simulink library "Lib_Piccolo"  (R2018b)
settings: Solver=VariableStepAuto  StartTime=0.0  StopTime=10.0  RelTol=1e-3
values from neighbouring files (symbols this model uses):
  AccelErrInt2Brakes = 0.15    [SimulationControlConfig16P.m]    (also in SimulationControlConfig16P_LEGACY.m; SimulationControlConfigTAILLESS.m = 0.2; SimulationControlConfigUTAIL.m = 0.2)
  AileronMax = 25    [SimulationControlConfig16P.m]    (also in SimulationControlConfig16P_LEGACY.m; SimulationControlConfigTAILLESS.m; SimulationControlConfigUTAIL.m)
  AileronPower = 0.00268    [SimulationControlConfig16P.m]    (also in SimulationControlConfig16P_LEGACY.m; SimulationControlConfigTAILLESS.m; SimulationControlConfigUTAIL.m)
  AileronSurfaceMax = 45    [SimulationControlConfig16P.m]    (also in SimulationControlConfig16P_LEGACY.m)
  AileronTrim = 0    [SimulationControlConfig16P.m]    (also in SimulationControlConfig16P_LEGACY.m; SimulationControlConfigTAILLESS.m; SimulationControlConfigUTAIL.m)
  Alt = 1000 + TerrainHeight    [SimulationStateConfig.m]
  AltCruise_m = testPlans(testIndx).terrainElevation * 0.3048 + 200    [SimulationControlConfig16P.m]    (also in SimulationControlConfigTAILLESS.m = 1083; SimulationControlConfigUTAIL.m = testPlans(testIndx).terrainElevation * 0.3048 + 152)
  AltitudeRate2PitchCmdIntegratorInit = 0.1    [SimulationControlPre.m]
  AltMax = 10000    [SimulationControlConfig16P.m]    (also in SimulationControlConfig16P_LEGACY.m; SimulationControlConfigTAILLESS.m; SimulationControlConfigUTAIL.m)
  AltMaxAccel = 1.25    [SimulationControlConfig16P.m]    (also in SimulationControlConfig16P_LEGACY.m = 0.9; SimulationControlConfigTAILLESS.m = 1.7; SimulationControlConfigUTAIL.m = 2)
  AltMin = 0    [SimulationControlConfig16P.m]    (also in SimulationControlConfig16P_LEGACY.m; SimulationControlConfigTAILLESS.m; SimulationControlConfigUTAIL.m)
  AltRateCmd2Pitch = 0.50    (= 0.5)    [SimulationControlConfig16P.m]    (also in SimulationControlConfig16P_LEGACY.m = 0.6; SimulationControlConfigTAILLESS.m = 0.2; SimulationControlConfigUTAIL.m = 0.3)
  AltRateError2Pitch = 0.40    (= 0.4)    [SimulationControlConfig16P.m]    (also in SimulationControlConfig16P_LEGACY.m; SimulationControlConfigTAILLESS.m = 0.55; SimulationControlConfigUTAIL.m = 0.55)
  AltRateErrorInt2Pitch = 0.50    (= 0.5)    [SimulationControlConfig16P.m]    (also in SimulationControlConfig16P_LEGACY.m = 0.45; SimulationControlConfigTAILLESS.m; SimulationControlConfigUTAIL.m = 0.75)
  AltRateLpfCutOff = 3    [SimulationControlConfig16P.m]    (also in SimulationControlConfig16P_LEGACY.m; SimulationControlConfigTAILLESS.m = 2; SimulationControlConfigUTAIL.m = 2)
  AutoNosegear2Rudder = 26    [SimulationControlConfig16P.m]    (also in SimulationControlConfig16P_LEGACY.m; SimulationControlConfigTAILLESS.m = 25.2; SimulationControlConfigUTAIL.m = 14)
  b = 5.54    [SimulationControlConfig16P.m]    (also in SimulationControlConfig16P_LEGACY.m; SimulationControlConfigTAILLESS.m = 2.37; SimulationControlConfigUTAIL.m = 2.37)
  Bank2AileronIntegratorInit = 0    [SimulationControlPre.m]
  BankMax_User = BankMax_User/180*pi    (= 0.523598775598)    [SimulationControlConfig16P.m]    (also in SimulationControlConfig16P_LEGACY.m; SimulationControlConfigTAILLESS.m = 0.610865238198; SimulationControlConfigUTAIL.m = 0.628318530718)
  baseLegFlaps = 20    [SimulationControlConfig16P.m]    (also in SimulationControlConfig16P_LEGACY.m = 0; SimulationControlConfigTAILLESS.m = 15; SimulationControlConfigUTAIL.m = 10)
  C = GeneticOpt.C    [SimulationCostFunction.m]
  c = Sw/b    (= 0.841696750903)    [SimulationControlConfig16P.m]    (also in SimulationControlConfig16P_LEGACY.m; SimulationControlConfigTAILLESS.m = 0.354008438819; SimulationControlConfigUTAIL.m = 0.354008438819)
  cell2WheelFactorMG = 5.98    [SimulationSensorConfig16P_LEGACY.m]
  cell2WheelFactorNG = 1    [SimulationSensorConfig16P_LEGACY.m]
  cellSatMaxMG = 15000    [SimulationSensorConfig16P.m]    (also in SimulationSensorConfig16P_LEGACY.m; SimulationSensorConfigTAILLESS7P.m; SimulationSensorConfigUTAIL7P.m)
  cellSatMaxNG = 1000    [SimulationSensorConfig16P.m]    (also in SimulationSensorConfig16P_LEGACY.m; SimulationSensorConfigTAILLESS7P.m; SimulationSensorConfigUTAIL7P.m)
  cellSatMinMG = -15000    [SimulationSensorConfig16P.m]    (also in SimulationSensorConfig16P_LEGACY.m; SimulationSensorConfigTAILLESS7P.m; SimulationSensorConfigUTAIL7P.m)
  cellSatMinNG = -1000    [SimulationSensorConfig16P.m]    (also in SimulationSensorConfig16P_LEGACY.m; SimulationSensorConfigTAILLESS7P.m; SimulationSensorConfigUTAIL7P.m)
  CL_Limit = CL_Max    (= 0.54)    [SimulationControlConfig16P.m]    (also in SimulationControlConfig16P_LEGACY.m; SimulationControlConfigTAILLESS.m; SimulationControlConfigUTAIL.m = 0.53)
  CL_Max = 0.54    [SimulationControlConfig16P.m]    (also in SimulationControlConfig16P_LEGACY.m; SimulationControlConfigTAILLESS.m; SimulationControlConfigUTAIL.m = 0.53)
  CL_Max_Nom = 0.465    [SimulationControlConfig16P.m]    (also in SimulationControlConfig16P_LEGACY.m; SimulationControlConfigTAILLESS.m = 0.39; SimulationControlConfigUTAIL.m)
  CL_Min = 0    [SimulationControlConfig16P.m]    (also in SimulationControlConfig16P_LEGACY.m; SimulationControlConfigTAILLESS.m; SimulationControlConfigUTAIL.m)
  ClimbMaxFraction = 0.35    [SimulationControlConfig16P.m]    (also in SimulationControlConfig16P_LEGACY.m = 0.24; SimulationControlConfigTAILLESS.m = 0.19; SimulationControlConfigUTAIL.m = 0.21)
  ClimboutMaxBank = 7.0    (= 7)    [SimulationControlConfig16P.m]    (also in SimulationControlConfig16P_LEGACY.m; SimulationControlConfigTAILLESS.m = 5; SimulationControlConfigUTAIL.m)
  ClimboutTimer = 7.0    (= 7)    [SimulationControlConfig16P.m]    (also in SimulationControlConfig16P_LEGACY.m; SimulationControlConfigTAILLESS.m; SimulationControlConfigUTAIL.m)
  dCl_per_dFlap = 0.005581818    [SimulationControlConfig16P.m]    (also in SimulationControlConfig16P_LEGACY.m = 0; SimulationControlConfigTAILLESS.m = 0; SimulationControlConfigUTAIL.m = 0)
  DecelerationCmd = 3.1    [SimulationControlConfig16P.m]    (also in SimulationControlConfig16P_LEGACY.m; SimulationControlConfigTAILLESS.m = 0.1; SimulationControlConfigUTAIL.m = 0.1)
  DeRotateLogicEndTimer = abs((NoseDownLimit_Deg-1)/DeRotateRamp_Dps)    [SimulationControlConfig16P.m]    (also in SimulationControlConfig16P_LEGACY.m; SimulationControlConfigTAILLESS.m; SimulationControlConfigUTAIL.m)
  DeRotateLogicHoldNoseUpTimer = 0.1    [SimulationControlConfig16P.m]    (also in SimulationControlConfig16P_LEGACY.m; SimulationControlConfigTAILLESS.m; SimulationControlConfigUTAIL.m)
  DeRotateLogicTimerTimeout = 2    [SimulationControlConfig16P.m]    (also in SimulationControlConfig16P_LEGACY.m; SimulationControlConfigTAILLESS.m; SimulationControlConfigUTAIL.m)
  DeRotateLowerCmdSaturation = 0    [SimulationControlConfig16P.m]    (also in SimulationControlConfig16P_LEGACY.m; SimulationControlConfigTAILLESS.m; SimulationControlConfigUTAIL.m)
  DeRotateRamp_Dps = 3    [SimulationControlConfig16P.m]    (also in SimulationControlConfig16P_LEGACY.m; SimulationControlConfigTAILLESS.m = 8; SimulationControlConfigUTAIL.m = 8)
  DeRotateUpperCmdSaturation = 7    [SimulationControlConfig16P.m]    (also in SimulationControlConfig16P_LEGACY.m; SimulationControlConfigTAILLESS.m; SimulationControlConfigUTAIL.m)
  DescentMaxFraction = 0.22    [SimulationControlConfig16P.m]    (also in SimulationControlConfig16P_LEGACY.m = 0.2; SimulationControlConfigTAILLESS.m = 0.17; SimulationControlConfigUTAIL.m = 0.17)
  DesktopSimTerrainOffset_m = 0.406    [SimulationAircraftConfig.m]
  downwindFlaps = 0    [SimulationControlConfig16P.m]    (also in SimulationControlConfig16P_LEGACY.m; SimulationControlConfigTAILLESS.m; SimulationControlConfigUTAIL.m)
  DP_init = 0.5*1.225*V_init^2    [SimulationControlConfig16P.m]    (also in SimulationControlConfig16P_LEGACY.m; SimulationControlConfigTAILLESS.m; SimulationControlConfigUTAIL.m)
  dscNoiseMG = 1    [SimulationSensorConfig16P_LEGACY.m]
  dscNoiseNG = 0.25    [SimulationSensorConfig16P_LEGACY.m]
  DSCnumBits = 24    [SimulationSensorConfig16P.m]    (also in SimulationSensorConfig16P_LEGACY.m; SimulationSensorConfigTAILLESS7P.m; SimulationSensorConfigUTAIL7P.m)
  DSCRangeMaxMG = 15000    [SimulationSensorConfig16P.m]    (also in SimulationSensorConfig16P_LEGACY.m; SimulationSensorConfigTAILLESS7P.m; SimulationSensorConfigUTAIL7P.m)
  DSCRangeMaxNG = 1000    [SimulationSensorConfig16P.m]    (also in SimulationSensorConfig16P_LEGACY.m; SimulationSensorConfigTAILLESS7P.m; SimulationSensorConfigUTAIL7P.m)
  DSCRangeMinMG = -15000    [SimulationSensorConfig16P.m]    (also in SimulationSensorConfig16P_LEGACY.m; SimulationSensorConfigTAILLESS7P.m; SimulationSensorConfigUTAIL7P.m)
  DSCRangeMinNG = -1000    [SimulationSensorConfig16P.m]    (also in SimulationSensorConfig16P_LEGACY.m; SimulationSensorConfigTAILLESS7P.m; SimulationSensorConfigUTAIL7P.m)
  dt = DLLSim.dt    [SimulationTimeStep.m]    (also in SimulationTrim.m = 0.02)
  EarlyTouchdownThreshold = 3.0    (= 3)    [SimulationControlConfig16P.m]    (also in SimulationControlConfig16P_LEGACY.m; SimulationControlConfigTAILLESS.m = 2.2; SimulationControlConfigUTAIL.m = 2.5)
  ElevatorDeflectionRate = 15    [SimulationControlConfig16P.m]    (also in SimulationControlConfig16P_LEGACY.m = 12; SimulationControlConfigTAILLESS.m = 10; SimulationControlConfigUTAIL.m = 12)
  ElevatorMax = 25    [SimulationControlConfig16P.m]    (also in SimulationControlConfig16P_LEGACY.m; SimulationControlConfigTAILLESS.m; SimulationControlConfigUTAIL.m)
  ElevatorPower = -0.002209    [SimulationControlConfig16P.m]    (also in SimulationControlConfig16P_LEGACY.m; SimulationControlConfigTAILLESS.m = -0.002956; SimulationControlConfigUTAIL.m = -0.00205983)
  ElevatorTrim = -3.5    [SimulationControlConfig16P.m]    (also in SimulationControlConfig16P_LEGACY.m; SimulationControlConfigTAILLESS.m = -6; SimulationControlConfigUTAIL.m = -8)
  elevonBias = 0    [SimulationControlConfig16P.m]    (also in SimulationControlConfig16P_LEGACY.m; SimulationControlConfigTAILLESS.m; SimulationControlConfigUTAIL.m)
  Enable_TAS_Protection = 0    [SimulationControlConfig16P.m]    (also in SimulationControlConfig16P_LEGACY.m; SimulationControlConfigTAILLESS.m; SimulationControlConfigUTAIL.m)
  EnableCrossTrackAbort = 1    [SimulationControlConfig16P.m]    (also in SimulationControlConfigTAILLESS.m; SimulationControlConfigUTAIL.m)
  EnergyBandwidth = 0.02    [SimulationControlConfig16P.m]    (also in SimulationControlConfig16P_LEGACY.m; SimulationControlConfigTAILLESS.m = 0.06; SimulationControlConfigUTAIL.m = 0.06)
  EngineLhFuelCut = 0    [SimulationAircraftConfig.m]
  EngineRhFuelCut = 0    [SimulationAircraftConfig.m]
  FastThrottleRate = 0.075    [SimulationControlConfig16P.m]    (also in SimulationControlConfig16P_LEGACY.m = 0.05; SimulationControlConfigTAILLESS.m = 0.1; SimulationControlConfigUTAIL.m = 0.1)
  FilterWarmUpTime = 2    [SimulationSensorConfig16P.m]    (also in SimulationSensorConfig16P_LEGACY.m; SimulationSensorConfigTAILLESS7P.m; SimulationSensorConfigUTAIL7P.m)
  finalApproachFlaps = 20    [SimulationControlConfig16P.m]    (also in SimulationControlConfig16P_LEGACY.m = 0; SimulationControlConfigTAILLESS.m = 22; SimulationControlConfigUTAIL.m = 10)
  FinalDescentSlope_Deg = testPlans(testIndx).descentSlope    [SimulationControlConfig16P.m]    (also in SimulationControlConfig16P_LEGACY.m; SimulationControlConfigTAILLESS.m; SimulationControlConfigUTAIL.m)
  flapMax = 0    [SimulationControlConfig16P.m]    (also in SimulationControlConfig16P_LEGACY.m; SimulationControlConfigTAILLESS.m; SimulationControlConfigUTAIL.m)
  flapRate = 7.5    [SimulationControlConfig16P.m]    (also in SimulationControlConfig16P_LEGACY.m; SimulationControlConfigTAILLESS.m = 6.6; SimulationControlConfigUTAIL.m)
  FlareHeight = 5    [SimulationControlConfig16P.m]    (also in SimulationControlConfig16P_LEGACY.m = 4.8; SimulationControlConfigTAILLESS.m = 2.5; SimulationControlConfigUTAIL.m = 2)
  FlareVerticalRate_mps = -0.4    [SimulationControlConfig16P.m]    (also in SimulationControlConfig16P_LEGACY.m = -0.5; SimulationControlConfigTAILLESS.m = -0.15; SimulationControlConfigUTAIL.m = -0.15)
  Fp_Aileron = 0.55*2*pi*RollRateLpfCutoff*dt    [SimulationControlConfig16P.m]    (also in SimulationControlConfig16P_LEGACY.m; SimulationControlConfigTAILLESS.m; SimulationControlConfigUTAIL.m)
  Fp_Alt = 0.55*AltBandwidth    (= 0.099)    [SimulationControlConfig16P.m]    (also in SimulationControlConfig16P_LEGACY.m; SimulationControlConfigTAILLESS.m = 0.587477826221; SimulationControlConfigUTAIL.m = 0.69115038379)
  Fp_AltRate = 0.55*2*pi*AltRateLpfCutOff*dt    [SimulationControlConfig16P.m]    (also in SimulationControlConfig16P_LEGACY.m; SimulationControlConfigTAILLESS.m; SimulationControlConfigUTAIL.m)
  Fp_Elevator = 0.55*2*pi*PitchRateLpfCutoff*dt    [SimulationControlConfig16P.m]    (also in SimulationControlConfig16P_LEGACY.m; SimulationControlConfigTAILLESS.m; SimulationControlConfigUTAIL.m)
  Fp_Energy = 0.55*2*pi*EnergyBandwidth    (= 0.069115038379)    [SimulationControlConfig16P.m]    (also in SimulationControlConfig16P_LEGACY.m; SimulationControlConfigTAILLESS.m = 0.207345115137; SimulationControlConfigUTAIL.m = 0.207345115137)
  Fp_Energy2 = 0.55*2*pi*EnergyBandwidth*dt    [SimulationControlConfig16P.m]    (also in SimulationControlConfig16P_LEGACY.m; SimulationControlConfigTAILLESS.m; SimulationControlConfigUTAIL.m)
  Fp_Pitch = 0.55*2*pi*PitchBandwidth    (= 2.76460153516)    [SimulationControlConfig16P.m]    (also in SimulationControlConfig16P_LEGACY.m = 3.11017672705; SimulationControlConfigTAILLESS.m = 3.80132711084; SimulationControlConfigUTAIL.m = 2.41902634326)
  Fp_Pitch_2 = 0.55*2*pi*PitchBandwidth*dt    [SimulationControlConfig16P.m]    (also in SimulationControlConfig16P_LEGACY.m; SimulationControlConfigTAILLESS.m; SimulationControlConfigUTAIL.m)
  Fp_Roll = RollBandwidth^2    (= 1)    [SimulationControlConfig16P.m]    (also in SimulationControlConfig16P_LEGACY.m = 1.44; SimulationControlConfigTAILLESS.m; SimulationControlConfigUTAIL.m)
  Fp_Rudder = 0.55*2*pi*YawRateLpfCutoff*dt    [SimulationControlConfig16P.m]    (also in SimulationControlConfig16P_LEGACY.m; SimulationControlConfigTAILLESS.m; SimulationControlConfigUTAIL.m)
  Fp_TAS = 0.55*2*pi*TASBandwidth    (= 0.103672557568)    [SimulationControlConfig16P.m]    (also in SimulationControlConfig16P_LEGACY.m; SimulationControlConfigTAILLESS.m = 0.172787595947; SimulationControlConfigUTAIL.m = 0.172787595947)
  Fp_TAS_Filter = 2*pi*TasLpfCutoff*dt    [SimulationControlConfig16P.m]    (also in SimulationControlConfig16P_LEGACY.m; SimulationControlConfigTAILLESS.m; SimulationControlConfigUTAIL.m)
  Fp_Turn = 0.55*2*pi*TurnErrLPFcutoff    (= 0.0345575191895)    [SimulationControlConfig16P.m]    (also in SimulationControlConfig16P_LEGACY.m; SimulationControlConfigTAILLESS.m = 0.172787595947; SimulationControlConfigUTAIL.m = 0.172787595947)
  Fp_TurnDerr = 0.55*2*pi*TurnDerivativeLPFcutoff    (= 0.0345575191895)    [SimulationControlConfig16P.m]    (also in SimulationControlConfig16P_LEGACY.m; SimulationControlConfigTAILLESS.m = 0.172787595947; SimulationControlConfigUTAIL.m = 0.172787595947)
  FTV = 3    [SimulationAircraftConfig.m]
  ftvStaticPositionError = 1/1.18    (= 0.847457627119)    [SimulationSensorConfig16P.m]    (also in SimulationSensorConfig16P_LEGACY.m; SimulationSensorConfigTAILLESS7P.m = 1; SimulationSensorConfigUTAIL7P.m = 1)
  g = 9.81    [SimulationStateConfig.m]
  GustSpd_Kts = testPlans(testIndx).gustSpd    [SimulationStateConfig.m]
  GustTriggerVal = testPlans(testIndx).gustTriggerVal    [SimulationStateConfig.m]
  HeadingErr2TurnRate = 0.5    [SimulationControlConfig16P.m]    (also in SimulationControlConfig16P_LEGACY.m; SimulationControlConfigTAILLESS.m; SimulationControlConfigUTAIL.m)
  HeadingErrDer2TurnRate = 0.3    [SimulationControlConfig16P.m]    (also in SimulationControlConfig16P_LEGACY.m; SimulationControlConfigTAILLESS.m; SimulationControlConfigUTAIL.m)
  IASbounce = IASstall*0.8    [SimulationControlPre.m]
  IAScruiseCMD = sqrt(2*m*9.81/(1.225*Sw*CL_cruise))    [SimulationControlConfig16P.m]    (also in SimulationControlConfig16P_LEGACY.m; SimulationControlConfigTAILLESS.m; SimulationControlConfigUTAIL.m)
  IASfinalCMD = 1.12 * IASmin    [SimulationControlConfig16P.m]    (also in SimulationControlConfig16P_LEGACY.m = 1.10 * IASmin; SimulationControlConfigTAILLESS.m = 1.10 * IASmin; SimulationControlConfigUTAIL.m = 1.15 * IASmin)
  IASflareCMD = IASstall    [SimulationControlConfig16P.m]    (also in SimulationControlConfig16P_LEGACY.m; SimulationControlConfigTAILLESS.m; SimulationControlConfigUTAIL.m)
  IASmax = 64    [SimulationControlConfig16P.m]    (also in SimulationControlConfig16P_LEGACY.m = 46; SimulationControlConfigTAILLESS.m = 38.58; SimulationControlConfigUTAIL.m = 35)
  IASmin = sqrt(2*m*9.81/(1.225*Sw*0.9*CL_Max_Nom))    [SimulationControlConfig16P.m]    (also in SimulationControlConfig16P_LEGACY.m; SimulationControlConfigTAILLESS.m; SimulationControlConfigUTAIL.m)
  IASshortCMD = IASstall    [SimulationControlConfig16P.m]    (also in SimulationControlConfig16P_LEGACY.m; SimulationControlConfigTAILLESS.m; SimulationControlConfigUTAIL.m)
  IASstall = sqrt(2*m*9.81/(1.225*Sw*CL_Max))    [SimulationControlConfig16P.m]    (also in SimulationControlConfig16P_LEGACY.m; SimulationControlConfigTAILLESS.m; SimulationControlConfigUTAIL.m)
  inFlight = 1    [SimulationControlConfig16P.m]    (also in SimulationControlConfigTAILLESS.m; SimulationControlConfigUTAIL.m)
  JetCatOffset = 5    [SimulationControlConfig16P.m]    (also in SimulationControlConfig16P_LEGACY.m)
  LaunchRollingElevator = -1.5    [SimulationControlConfig16P.m]    (also in SimulationControlConfig16P_LEGACY.m; SimulationControlConfigTAILLESS.m = 1; SimulationControlConfigUTAIL.m = 1)
  ldg_NosegearMax = 10    [SimulationControlConfig16P.m]    (also in SimulationControlConfig16P_LEGACY.m; SimulationControlConfigTAILLESS.m; SimulationControlConfigUTAIL.m)
  ldg_TrackVyErrInt2Nosegear = 0.1250    (= 0.125)    [SimulationControlConfig16P.m]    (also in SimulationControlConfig16P_LEGACY.m; SimulationControlConfigTAILLESS.m = 0.00714285714286; SimulationControlConfigUTAIL.m = 0.00714285714286)
  ldg_TrackVyErrPro2Nosegear = 0.35    [SimulationControlConfig16P.m]    (also in SimulationControlConfig16P_LEGACY.m; SimulationControlConfigTAILLESS.m = 0.0546666666667; SimulationControlConfigUTAIL.m = 0.0546666666667)
  ldg_TrackY2Vy = 0.07    [SimulationControlConfig16P.m]    (also in SimulationControlConfig16P_LEGACY.m; SimulationControlConfigTAILLESS.m = 0.17; SimulationControlConfigUTAIL.m = 0.17)
  ldg_Vy2NosegearScalingPower = 1.075    [SimulationControlConfig16P.m]    (also in SimulationControlConfig16P_LEGACY.m; SimulationControlConfigTAILLESS.m = 0.6; SimulationControlConfigUTAIL.m = 0.5)
  ldg_Y2VyScalingPower = 0.175    [SimulationControlConfig16P.m]    (also in SimulationControlConfig16P_LEGACY.m; SimulationControlConfigTAILLESS.m = 0; SimulationControlConfigUTAIL.m = 0)
  ldg_YawRate2Nosegear = 0.175    [SimulationControlConfig16P.m]    (also in SimulationControlConfig16P_LEGACY.m; SimulationControlConfigTAILLESS.m = 0.065; SimulationControlConfigUTAIL.m = 0.065)
  LiftSlope = 0.064285    [SimulationControlConfig16P.m]    (also in SimulationControlConfig16P_LEGACY.m; SimulationControlConfigTAILLESS.m = 0.058631; SimulationControlConfigUTAIL.m)
  LPFaileronInit = 0    [SimulationControlPre.m]
  LPFclestInit = 0    [SimulationControlPre.m]
  LPFenergyFFInit = 0    [SimulationControlPre.m]
  LPFtasInit = V_init + 2    [SimulationControlPre.m]
  LPFthrottleInit = ThrottleTrim    [SimulationControlPre.m]
  LPFturnErrInit = 0    [SimulationControlPre.m]
  ... (+115 more)
undefined symbols (not defined in the file or in its folder): abortFlag, alphaHPF, apmDelay, BRWNOUT, CRAWOR, CRAWUR, DiscIntNeverNeededParam, DLLSim, DLLSimStep, ECOMOR, ECOMUR, Fp_Tas, GustTrigger_HeightAgl_m, IPSTAT, LCINTEG, Ldg_Persist_Time, LOWER_FLAGS, MSG_ENABLE, NoiseStd, OLDVAL, OVERRIDE_ENABLE, OVERRIDE_VALUE, REBOOT, reversionEnable, revIASMax, revIASMin, revPitchMax, revPitchMin, revPitchRateMax, revRollMax, revRollRateMax, SAMPLE, SCALON, SensorModel, sigbuilder_block, Sim_Vx, Sim_Vy, Sim_Vz, Sim_Xpos, Sim_Ypos, Sim_Zpos, SYSOR, SYSUR, TARE, TEMPOR, TEMPUR, testIndx, testPlan, testPlans, Trim_piccoloInCmd, Trim_REFSI_FD_IN_nmodeCgShifterCmd_Ft, Trim_REFSI_FD_IN_nmodeFlapLhIBCmd_Deg, Trim_REFSI_FD_IN_nmodeFlapLhOBCmd_Deg, Trim_REFSI_FD_IN_nmodeFlapRhIBCmd_Deg, Trim_REFSI_FD_IN_nmodeFlapRhOBCmd_Deg, Trim_REFSI_FD_IN_nmodeSlatLhCmd_Deg, Trim_REFSI_FD_IN_nmodeSlatRhCmd_Deg, Trim_REFSI_FD_IN_nmodeSplrLhInbdCmd_Deg, Trim_REFSI_FD_IN_nmodeSplrLhOutbdCmd_Deg ... (+5)
libraries: simulink x866, aerolibconvert2 x60, $bdroot x52, aerolibatmos2 x5, dspswit3 x5, simulink_extras x4, dsparch4 x2, Lib_Piccolo_Alt x2, eeGeneralControl x1, dspindex x1
(part 6 of 44)

== system Lib_Piccolo/WOW Archive Container ==
  note: 15 - Landing logic matched to LOAD14, differs in takeoff:
      | - Ability to use Piccolo mode changes as analog for airspeed to drive weight-off-wheels signal
  note: 14 - Logic derived from LOAD2, with key changes:
      | - Saturation on inputs to filter to prevent 'wind-up'
  note: 17 - Landing logic matched to LOAD16, differs in takeoff:
      | - Ability to use Piccolo mode changes as analog for airspeed to drive weight-off-wheels signal
  Load Cell WoW Model 10 : Subsystem  VariantControl="SensorModel.WOW.Cell.Variant==\"LOAD10\""
  Load Cell WoW Model 10_OLD : Subsystem  VariantControl="SensorModel.WOW.Cell.Variant==\"LOAD10_OLD\""
  Load Cell WoW Model 11 : Subsystem  VariantControl="SensorModel.WOW.Cell.Variant==\"LOAD11\""
  Load Cell WoW Model 11_OLD : Subsystem  VariantControl="SensorModel.WOW.Cell.Variant==\"LOAD11_OLD\""
  Load Cell WoW Model 12 : Subsystem  VariantControl="SensorModel.WOW.Cell.Variant==\"LOAD12\""
  Load Cell WoW Model 14 : Subsystem  VariantControl="SensorModel.WOW.Cell.Variant==\"LOAD14\""
  Load Cell WoW Model 15 : Subsystem  VariantControl="SensorModel.WOW.Cell.Variant==\"LOAD15\""
  Load Cell WoW Model 17 : Subsystem  VariantControl="SensorModel.WOW.Cell.Variant==\"LOAD17\""
  Load Cell WoW Model 2 : Subsystem  VariantControl="SensorModel.WOW.Cell.Variant==\"LOAD2\""
  Load Cell WoW Model 3 - LiftOff Delay : Subsystem  VariantControl="SensorModel.WOW.Cell.Variant==\"LOAD3\""  mask{Ldg_Persist_Time=SensorModel.WOW.Cell.persistanceTime_s, Ldg_Latch_Time_P=SensorModel.WOW.Cell.longLatchTime_s, Ldg_Latch_Time_S=SensorModel.WOW.Cell.shortLatchTime_s, Ldg_Load_Thresh_Upper=SensorModel.WOW.Cell.loadThresholdUpper_N, Ldg_Load_Thresh_Lower=SensorModel.WOW.Cell.loadThresholdLower_N, TO_Persist_Time=SensorModel.WOW.Cell.TO_persistanceTime_s, TO_Latch_Time=SensorModel.WOW.Cell.TO_latchTime_s, TO_Load_Thresh=SensorModel.WOW.Cell.TO_loadThreshold_N, DSCnumBits=24, numBits=16, satMaxMG=15000, satMinMG=-300, dscNoiseMG=1, DSCRangeMaxMG=15000, DSCRangeMinMG=-15000, satMaxNG=1000, satMinNG=-250, dscNoiseNG=0.25, DSCRangeMaxNG=1000, DSCRangeMinNG=-1000, cellSatMaxMG=15000, cellSatMinMG=-15000, cell2WheelFactorMG=5.98, cellSatMaxNG=1000, cellSatMinNG=-1000, cell2WheelFactorNG=1}
      mask prompts: Ldg_Persist_Time "Landing Persistance Time [s]"; Ldg_Latch_Time_P "Primary Landing Latch Time [s]"; Ldg_Latch_Time_S "Secondary Landing Latch Time [s]"; Ldg_Load_Thresh_Upper "Landing Load Threshold Upper [N]"; Ldg_Load_Thresh_Lower "Landing Load Threshold Lower [N]"; TO_Persist_Time "Take Off Persistance Time [s]"; TO_Latch_Time "Take Off Latch Time [s]"; TO_Load_Thresh "Take Off Load Threshold  [N]"; DSCnumBits "DSC Encoded Resolution [num bits]"; numBits "CANBridge Encoded Resolution [num bits]"; satMaxMG "Main Gear CANBridge Saturation Max [N]"; satMinMG "Main Gear CANBridge Saturation Min [N]"; dscNoiseMG "Main Gear DSC Noise Level pk-pk [N]"; DSCRangeMaxMG "Main Gear DSC Range Max [N]"; DSCRangeMinMG "Main Gear DSC Range Min [N]"; satMaxNG "Nose Gear CANBridge Saturation Max [N]"; satMinNG "Nose Gear CANBridge Saturation Min [N]"; dscNoiseNG "Nose Gear DSC Noise Level pk-pk [N]"; DSCRangeMaxNG "Nose Gear DSC Range Max [N]"; DSCRangeMinNG "Nose Gear DSC Range Min [N]"; cellSatMaxMG "Main Gear Cell Saturation Max [N]"; cellSatMinMG "Main Gear Cell Saturation Min [N]"; cell2WheelFactorMG "Main Gear Cell to Wheel Load Scale Factor"; cellSatMaxNG "Nose Gear Cell Saturation Max [N]"; cellSatMinNG "Nose Gear Cell Saturation Min [N]"; cell2WheelFactorNG "Nose Gear Cell to Wheel Load Scale Factor"
      mask DialogControl DescGroupVar Prompt: Full model of load-cell based weight-on-wheels system.
      mask DialogControl LogicGroupVar Prompt: Logic Configuration
      mask DialogControl DataGroupVar Prompt: Data Acquisition
      mask DialogControl Container5 Prompt: MG
      mask DialogControl Container6 Prompt: NG
      mask DialogControl ParamGroupVar Prompt: Physical Parameters
      mask DialogControl Container8 Prompt: MG
      mask DialogControl Container9 Prompt: NG
  Load Cell WoW Model 4 - LiftOff Delay variation 2 : Subsystem  VariantControl="SensorModel.WOW.Cell.Variant==\"LOAD4\""  mask{Ldg_Persist_Time=SensorModel.WOW.Cell.persistanceTime_s, Ldg_Latch_Time_P=SensorModel.WOW.Cell.longLatchTime_s, Ldg_Latch_Time_S=SensorModel.WOW.Cell.shortLatchTime_s, Ldg_Load_Thresh_Upper=SensorModel.WOW.Cell.loadThresholdUpper_N, Ldg_Load_Thresh_Lower=SensorModel.WOW.Cell.loadThresholdLower_N, TO_Persist_Time=SensorModel.WOW.Cell.TO_persistanceTime_s, TO_Latch_Time=SensorModel.WOW.Cell.TO_latchTime_s, TO_Load_Thresh=SensorModel.WOW.Cell.TO_loadThreshold_N, DSCnumBits=24, numBits=16, satMaxMG=15000, satMinMG=-300, dscNoiseMG=1, DSCRangeMaxMG=15000, DSCRangeMinMG=-15000, satMaxNG=1000, satMinNG=-250, dscNoiseNG=0.25, DSCRangeMaxNG=1000, DSCRangeMinNG=-1000, cellSatMaxMG=15000, cellSatMinMG=-15000, cell2WheelFactorMG=5.98, cellSatMaxNG=1000, cellSatMinNG=-1000, cell2WheelFactorNG=1}
      mask prompts: Ldg_Persist_Time "Landing Persistance Time [s]"; Ldg_Latch_Time_P "Primary Landing Latch Time [s]"; Ldg_Latch_Time_S "Secondary Landing Latch Time [s]"; Ldg_Load_Thresh_Upper "Landing Load Threshold Upper [N]"; Ldg_Load_Thresh_Lower "Landing Load Threshold Lower [N]"; TO_Persist_Time "Take Off Persistance Time [s]"; TO_Latch_Time "Take Off Latch Time [s]"; TO_Load_Thresh "Take Off Load Threshold  [N]"; DSCnumBits "DSC Encoded Resolution [num bits]"; numBits "CANBridge Encoded Resolution [num bits]"; satMaxMG "Main Gear CANBridge Saturation Max [N]"; satMinMG "Main Gear CANBridge Saturation Min [N]"; dscNoiseMG "Main Gear DSC Noise Level pk-pk [N]"; DSCRangeMaxMG "Main Gear DSC Range Max [N]"; DSCRangeMinMG "Main Gear DSC Range Min [N]"; satMaxNG "Nose Gear CANBridge Saturation Max [N]"; satMinNG "Nose Gear CANBridge Saturation Min [N]"; dscNoiseNG "Nose Gear DSC Noise Level pk-pk [N]"; DSCRangeMaxNG "Nose Gear DSC Range Max [N]"; DSCRangeMinNG "Nose Gear DSC Range Min [N]"; cellSatMaxMG "Main Gear Cell Saturation Max [N]"; cellSatMinMG "Main Gear Cell Saturation Min [N]"; cell2WheelFactorMG "Main Gear Cell to Wheel Load Scale Factor"; cellSatMaxNG "Nose Gear Cell Saturation Max [N]"; cellSatMinNG "Nose Gear Cell Saturation Min [N]"; cell2WheelFactorNG "Nose Gear Cell to Wheel Load Scale Factor"
      mask DialogControl DescGroupVar Prompt: Full model of load-cell based weight-on-wheels system.
      mask DialogControl LogicGroupVar Prompt: Logic Configuration
      mask DialogControl DataGroupVar Prompt: Data Acquisition
      mask DialogControl Container5 Prompt: MG
      mask DialogControl Container6 Prompt: NG
      mask DialogControl ParamGroupVar Prompt: Physical Parameters
      mask DialogControl Container8 Prompt: MG
      mask DialogControl Container9 Prompt: NG
  Load Cell WoW Model 5 - Dynamic Timing : Subsystem  VariantControl="SensorModel.WOW.Cell.Variant==\"LOAD5\""  mask{Ldg_Persist_Time=SensorModel.WOW.Cell.persistanceTime_s, Ldg_Latch_Time_P=SensorModel.WOW.Cell.longLatchTime_s, Ldg_Latch_Time_S=SensorModel.WOW.Cell.shortLatchTime_s, Ldg_Load_Thresh_Upper=SensorModel.WOW.Cell.loadThresholdUpper_N, Ldg_Load_Thresh_Lower=SensorModel.WOW.Cell.loadThresholdLower_N, TO_Persist_Time=SensorModel.WOW.Cell.TO_persistanceTime_s, TO_Latch_Time=SensorModel.WOW.Cell.TO_latchTime_s, TO_Load_Thresh=SensorModel.WOW.Cell.TO_loadThreshold_N, DSCnumBits=24, numBits=16, satMaxMG=15000, satMinMG=-300, dscNoiseMG=1, DSCRangeMaxMG=15000, DSCRangeMinMG=-15000, satMaxNG=1000, satMinNG=-250, dscNoiseNG=0.25, DSCRangeMaxNG=1000, DSCRangeMinNG=-1000, cellSatMaxMG=15000, cellSatMinMG=-15000, cell2WheelFactorMG=5.98, cellSatMaxNG=1000, cellSatMinNG=-1000, cell2WheelFactorNG=1}
      mask prompts: Ldg_Persist_Time "Landing Persistance Time [s]"; Ldg_Latch_Time_P "Primary Landing Latch Time [s]"; Ldg_Latch_Time_S "Secondary Landing Latch Time [s]"; Ldg_Load_Thresh_Upper "Landing Load Threshold Upper [N]"; Ldg_Load_Thresh_Lower "Landing Load Threshold Lower [N]"; TO_Persist_Time "Take Off Persistance Time [s]"; TO_Latch_Time "Take Off Latch Time [s]"; TO_Load_Thresh "Take Off Load Threshold  [N]"; DSCnumBits "DSC Encoded Resolution [num bits]"; numBits "CANBridge Encoded Resolution [num bits]"; satMaxMG "Main Gear CANBridge Saturation Max [N]"; satMinMG "Main Gear CANBridge Saturation Min [N]"; dscNoiseMG "Main Gear DSC Noise Level pk-pk [N]"; DSCRangeMaxMG "Main Gear DSC Range Max [N]"; DSCRangeMinMG "Main Gear DSC Range Min [N]"; satMaxNG "Nose Gear CANBridge Saturation Max [N]"; satMinNG "Nose Gear CANBridge Saturation Min [N]"; dscNoiseNG "Nose Gear DSC Noise Level pk-pk [N]"; DSCRangeMaxNG "Nose Gear DSC Range Max [N]"; DSCRangeMinNG "Nose Gear DSC Range Min [N]"; cellSatMaxMG "Main Gear Cell Saturation Max [N]"; cellSatMinMG "Main Gear Cell Saturation Min [N]"; cell2WheelFactorMG "Main Gear Cell to Wheel Load Scale Factor"; cellSatMaxNG "Nose Gear Cell Saturation Max [N]"; cellSatMinNG "Nose Gear Cell Saturation Min [N]"; cell2WheelFactorNG "Nose Gear Cell to Wheel Load Scale Factor"
      mask DialogControl DescGroupVar Prompt: Full model of load-cell based weight-on-wheels system.
      mask DialogControl LogicGroupVar Prompt: Logic Configuration
      mask DialogControl DataGroupVar Prompt: Data Acquisition
      mask DialogControl Container5 Prompt: MG
      mask DialogControl Container6 Prompt: NG
      mask DialogControl ParamGroupVar Prompt: Physical Parameters
      mask DialogControl Container8 Prompt: MG
      mask DialogControl Container9 Prompt: NG
  Load Cell WoW Model 6 - LiftOff Delay variation 3 : Subsystem  VariantControl="SensorModel.WOW.Cell.Variant==\"LOAD6\""  mask{Ldg_Persist_Time=SensorModel.WOW.Cell.persistanceTime_s, Ldg_Latch_Time_P=SensorModel.WOW.Cell.longLatchTime_s, Ldg_Latch_Time_S=SensorModel.WOW.Cell.shortLatchTime_s, Ldg_Load_Thresh_Upper=SensorModel.WOW.Cell.loadThresholdUpper_N, Ldg_Load_Thresh_Lower=SensorModel.WOW.Cell.loadThresholdLower_N, TO_Persist_Time=SensorModel.WOW.Cell.TO_persistanceTime_s, TO_Latch_Time=SensorModel.WOW.Cell.TO_latchTime_s, TO_Load_Thresh=SensorModel.WOW.Cell.TO_loadThreshold_N, DSCnumBits=24, numBits=16, satMaxMG=15000, satMinMG=-300, dscNoiseMG=1, DSCRangeMaxMG=15000, DSCRangeMinMG=-15000, satMaxNG=1000, satMinNG=-250, dscNoiseNG=0.25, DSCRangeMaxNG=1000, DSCRangeMinNG=-1000, cellSatMaxMG=15000, cellSatMinMG=-15000, cell2WheelFactorMG=5.98, cellSatMaxNG=1000, cellSatMinNG=-1000, cell2WheelFactorNG=1}
      mask prompts: Ldg_Persist_Time "Landing Persistance Time [s]"; Ldg_Latch_Time_P "Primary Landing Latch Time [s]"; Ldg_Latch_Time_S "Secondary Landing Latch Time [s]"; Ldg_Load_Thresh_Upper "Landing Load Threshold Upper [N]"; Ldg_Load_Thresh_Lower "Landing Load Threshold Lower [N]"; TO_Persist_Time "Take Off Persistance Time [s]"; TO_Latch_Time "Take Off Latch Time [s]"; TO_Load_Thresh "Take Off Load Threshold  [N]"; DSCnumBits "DSC Encoded Resolution [num bits]"; numBits "CANBridge Encoded Resolution [num bits]"; satMaxMG "Main Gear CANBridge Saturation Max [N]"; satMinMG "Main Gear CANBridge Saturation Min [N]"; dscNoiseMG "Main Gear DSC Noise Level pk-pk [N]"; DSCRangeMaxMG "Main Gear DSC Range Max [N]"; DSCRangeMinMG "Main Gear DSC Range Min [N]"; satMaxNG "Nose Gear CANBridge Saturation Max [N]"; satMinNG "Nose Gear CANBridge Saturation Min [N]"; dscNoiseNG "Nose Gear DSC Noise Level pk-pk [N]"; DSCRangeMaxNG "Nose Gear DSC Range Max [N]"; DSCRangeMinNG "Nose Gear DSC Range Min [N]"; cellSatMaxMG "Main Gear Cell Saturation Max [N]"; cellSatMinMG "Main Gear Cell Saturation Min [N]"; cell2WheelFactorMG "Main Gear Cell to Wheel Load Scale Factor"; cellSatMaxNG "Nose Gear Cell Saturation Max [N]"; cellSatMinNG "Nose Gear Cell Saturation Min [N]"; cell2WheelFactorNG "Nose Gear Cell to Wheel Load Scale Factor"
      mask DialogControl DescGroupVar Prompt: Full model of load-cell based weight-on-wheels system.
      mask DialogControl LogicGroupVar Prompt: Logic Configuration
      mask DialogControl DataGroupVar Prompt: Data Acquisition
      mask DialogControl Container5 Prompt: MG
      mask DialogControl Container6 Prompt: NG
      mask DialogControl ParamGroupVar Prompt: Physical Parameters
      mask DialogControl Container8 Prompt: MG
      mask DialogControl Container9 Prompt: NG
  Load Cell WoW Model 7 - LiftOff Delay variation 4 : Subsystem  VariantControl="SensorModel.WOW.Cell.Variant==\"LOAD7\""  mask{Ldg_Persist_Time=SensorModel.WOW.Cell.persistanceTime_s, Ldg_Latch_Time_P=SensorModel.WOW.Cell.longLatchTime_s, Ldg_Latch_Time_S=SensorModel.WOW.Cell.shortLatchTime_s, Ldg_Load_Thresh_Upper=SensorModel.WOW.Cell.loadThresholdUpper_N, Ldg_Load_Thresh_Lower=SensorModel.WOW.Cell.loadThresholdLower_N, TO_Persist_Time=SensorModel.WOW.Cell.TO_persistanceTime_s, TO_Latch_Time=SensorModel.WOW.Cell.TO_latchTime_s, TO_Load_Thresh=SensorModel.WOW.Cell.TO_loadThreshold_N, DSCnumBits=24, numBits=16, satMaxMG=15000, satMinMG=-300, dscNoiseMG=1, DSCRangeMaxMG=15000, DSCRangeMinMG=-15000, satMaxNG=1000, satMinNG=-250, dscNoiseNG=0.25, DSCRangeMaxNG=1000, DSCRangeMinNG=-1000, cellSatMaxMG=15000, cellSatMinMG=-15000, cell2WheelFactorMG=5.98, cellSatMaxNG=1000, cellSatMinNG=-1000, cell2WheelFactorNG=1}
      mask prompts: Ldg_Persist_Time "Landing Persistance Time [s]"; Ldg_Latch_Time_P "Primary Landing Latch Time [s]"; Ldg_Latch_Time_S "Secondary Landing Latch Time [s]"; Ldg_Load_Thresh_Upper "Landing Load Threshold Upper [N]"; Ldg_Load_Thresh_Lower "Landing Load Threshold Lower [N]"; TO_Persist_Time "Take Off Persistance Time [s]"; TO_Latch_Time "Take Off Latch Time [s]"; TO_Load_Thresh "Take Off Load Threshold  [N]"; DSCnumBits "DSC Encoded Resolution [num bits]"; numBits "CANBridge Encoded Resolution [num bits]"; satMaxMG "Main Gear CANBridge Saturation Max [N]"; satMinMG "Main Gear CANBridge Saturation Min [N]"; dscNoiseMG "Main Gear DSC Noise Level pk-pk [N]"; DSCRangeMaxMG "Main Gear DSC Range Max [N]"; DSCRangeMinMG "Main Gear DSC Range Min [N]"; satMaxNG "Nose Gear CANBridge Saturation Max [N]"; satMinNG "Nose Gear CANBridge Saturation Min [N]"; dscNoiseNG "Nose Gear DSC Noise Level pk-pk [N]"; DSCRangeMaxNG "Nose Gear DSC Range Max [N]"; DSCRangeMinNG "Nose Gear DSC Range Min [N]"; cellSatMaxMG "Main Gear Cell Saturation Max [N]"; cellSatMinMG "Main Gear Cell Saturation Min [N]"; cell2WheelFactorMG "Main Gear Cell to Wheel Load Scale Factor"; cellSatMaxNG "Nose Gear Cell Saturation Max [N]"; cellSatMinNG "Nose Gear Cell Saturation Min [N]"; cell2WheelFactorNG "Nose Gear Cell to Wheel Load Scale Factor"
      mask DialogControl DescGroupVar Prompt: Full model of load-cell based weight-on-wheels system.
      mask DialogControl LogicGroupVar Prompt: Logic Configuration
      mask DialogControl DataGroupVar Prompt: Data Acquisition
      mask DialogControl Container5 Prompt: MG
      mask DialogControl Container6 Prompt: NG
      mask DialogControl ParamGroupVar Prompt: Physical Parameters
      mask DialogControl Container8 Prompt: MG
      mask DialogControl Container9 Prompt: NG
  Load Cell WoW Model 8 : Subsystem  VariantControl="SensorModel.WOW.Cell.Variant==\"LOAD8\""
  Load Cell WoW Model 9 : Subsystem  VariantControl="SensorModel.WOW.Cell.Variant==\"LOAD9\""

== system Lib_Piccolo/Yaw to Rudder ==
  note: Filtering, Trim & Pilot Injection
  note: Kinematic Yaw Rate Coordination
  note: Coordintation Control Mode Selection
  note: Side-Force Integration Coordination
  note: Yaw Damping
  SideSlipCmd : Inport
  Feedback Bus : Inport  Port=2
  Bus Selector : BusSelector  OutputSignals=yAccel_Body_mps2,Roll_Euler_rad,V_mps,YawRate_Body_radps,DynamicPressure_Pa
  Compare To Constant : simulink/Logic and Bit Operations/Compare To Constant  relop=<=  const=2  OutDataTypeStr=boolean
  Compare To Constant1 : simulink/Logic and Bit Operations/Compare To Constant  relop=>  const=0  OutDataTypeStr=uint8
  Compare To Constant2 : simulink/Logic and Bit Operations/Compare To Constant  relop=>=  const=11  OutDataTypeStr=boolean
  Constant : Constant  Value=g
  Constant1 : Constant  Value=Sw
  Constant10 : Constant  Value=SideForceErrInt2Rudder
  Constant11 : Constant  Value=RudderTrim
  Constant2 : Constant  Value=b
  Constant3 : Constant  Value=RudderPower
  Constant4 : Constant  Value=m
  Constant5 : Constant  Value=Sw
  Constant6 : Constant  Value=RudderEffect
  Constant7 : Constant  Value=SideslipEffect
  Constant8 : Constant  Value=Yaw2RudderSideForceIntegratorInit
  Controller Selection : Subsystem
  Discrete-Time Integrator1 : DiscreteIntegrator  IntegratorMethod=Integration: Backward Euler  ExternalReset=falling  InitialConditionSource=external  SampleTime=-1  LimitOutput=on  UpperSaturationLimit=RudderMax  LowerSaturationLimit=-RudderMax  ICPrevOutput=DiscIntNeverNeededParam  ICPrevScaledInput=DiscIntNeverNeededParam
  Gain : Gain  Gain=-1
  Gain2 : Gain  Gain=180/pi
  KI_SideForce : Gain  Gain=SideForceErrInt2Rudder
  LPF RudderCmd : Subsystem
  Max : MinMax  Function=max  Inputs=2
  Multiply : Product  Inputs=**/
  Multiply1 : Product  Inputs=**/
  Multiply2 : Product  Inputs=*/
  Multiply3 : Product  Inputs=***////
  Multiply4 : Product  Inputs=**////
  NOT : Logic  Operator=NOT  IconShape=distinctive  AllPortsSameDT=off  OutDataTypeStr=boolean
  OR : Logic  Operator=OR  IconShape=distinctive  AllPortsSameDT=off  OutDataTypeStr=boolean
  Pilot Rudder : Subsystem
  "Rad to Deg " : Gain  Gain=180/pi
  RudderEffect : Constant  Value=RudderEffect
  Saturation : Saturate  UpperLimit=RudderMax  LowerLimit=-RudderMax
  Saturation2 : Saturate  UpperLimit=RudderMax  LowerLimit=-RudderMax
  Sin : Trigonometry
  Sum : Sum  Inputs=-+|
  Sum1 : Sum  Inputs=|++
  Sum2 : Sum  Inputs=+++
  Switch : Switch  Criteria=u2 > Threshold
  Switch2 : Switch  Criteria=u2 > Threshold  Threshold=0.5
  Terminator : Terminator
  Terminator1 : Terminator
  Use V_Lim : Gain
  VerticalTailArm : Constant  Value=VerticalTailArm
  YawRateErr2Rudder : Constant  Value=YawRateErr2Rudder
  Z inertia : Constant  Value=ZInertia
  Rudder_Deg : Outport
  tag scope: Coord_Rud=global
  wires:
  Switch2/1 -> LPF RudderCmd/1(Input)
  NOT/1 -> LPF RudderCmd/2(Reset)
  [ApGlobal] -> NOT/1, Switch2/2
  [pilotRud] -> LPF RudderCmd/3(ResetValue), Switch2/3
  Feedback Bus/1 -> Bus Selector/1
  Bus Selector/2 -> Sin/1  "<Roll_Euler_rad>"
  Bus Selector/3 -> Use V_Lim/1  "<V_mps>"
  Bus Selector/5 -> Multiply4/3, Max/1  "<DynamicPressure_Pa>"
  Sin/1 -> Multiply/2
  Constant/1 -> Multiply/1
  Use V_Lim/1 -> Multiply1/3, Multiply/3  "Sim.TAS"
  Multiply/1 -> Multiply1/2, Gain2/1, Sum/1  "YawRate_Desired"
  VerticalTailArm/1 -> Multiply1/1
  Multiply1/1 -> Multiply2/1  "Sideslip angle (Beta)"
  RudderEffect/1 -> Multiply2/2
  Multiply2/1 -> "Rad to Deg "/1
  Bus Selector/4 -> Sum/2  "<YawRate_Body_radps>"
  [Qmin] -> Max/2
  YawRateErr2Rudder/1 -> Multiply3/1
  Sum/1 -> Multiply3/2
  Z inertia/1 -> Multiply3/3
  Max/1 -> Multiply3/4
  Constant1/1 -> Multiply3/5
  Constant2/1 -> Multiply3/6
  Constant3/1 -> Multiply3/7
  Multiply3/1 -> Sum1/2  "deltaRudder_Damping_Deg"
  Gain2/1 -> Terminator/1  "Sim.yawRateCmd"
  LPF RudderCmd/1(Output) -> Sum2/2
  Bus Selector/1 -> Multiply4/2  "<yAccel_Body_mps2>"
  Constant4/1 -> Multiply4/1
  Constant5/1 -> Multiply4/4
  Constant6/1 -> Multiply4/5
  Constant7/1 -> Multiply4/6
  Multiply4/1 -> KI_SideForce/1
  Saturation2/1 -> Switch/1  "deltaRudder_SideForce_Coordination_Deg"
  Switch/1 -> Sum1/1
  Constant10/1 -> Compare To Constant1/1
  Compare To Constant1/1 -> Switch/2
  Sum1/1 -> Gain/1
  KI_SideForce/1 -> Discrete-Time Integrator1/1
  Constant8/1 -> Discrete-Time Integrator1/3
  Controller Selection/1(Rudder Out) -> Rudder_Deg/1
  Sum2/1 -> Saturation/1
  Saturation/1 -> [Coord_Rud]
  Constant11/1 -> Sum2/3
  [Pic_AP_Mode] -> Compare To Constant2/1, Compare To Constant/1
  Compare To Constant/1 -> OR/1
  Compare To Constant2/1 -> OR/2
  OR/1 -> Discrete-Time Integrator1/2  "sideForceIntReset"
  Discrete-Time Integrator1/1 -> Saturation2/1
  "Rad to Deg "/1 -> Switch/3  "deltaRudder_Coordination_Deg"
  Gain/1 -> Switch2/1
  SideSlipCmd/1 -> Terminator1/1
  Pilot Rudder/1(Rudder Out) -> Sum2/1

== system Lib_Piccolo/ Dynamic Timer/Enabled Subsystem ==
  periodIn : Inport
  Enable : EnablePort
  Gain : Gain
  periodOut : Outport
  wires:
  periodIn/1 -> Gain/1
  Gain/1 -> periodOut/1

== system Lib_Piccolo/A//C Dynamics/DLLSimulation ==
  SimInputBus : Inport
  Bus to Vector : BusToVector
  Bus2Vect2 : Subsystem  Commented=on
      mask init:
      | CurrentSys = gcs;
      | blockName = get_param(gcb,'Name');
      | 
      | CurBlk = [CurrentSys,'/',blockName];%Current block
      | BusSel = [CurrentSys,'/',blockName,'/BusSelector'];%BusSelectorBlock
      | BusMux = [CurrentSys,'/',blockName,'/Mux'];%Mux bloxk
      | 
      | 
      | 
      | Inputs = get_param(BusSel,'InputSignals');
      | 
      | 
      | outsig='';
      | for i=1:length(Inputs)
      |     outsig=[outsig Inputs{i} ','];
      | end;
      | outsig=outsig(1:length(outsig)-1);
      | 
      |     for nnn = 1:str2double(get_param(BusMux,'Inputs'))
      |         delete_line([CurrentSys '/' blockName],['BusSelector/' num2str(nnn)],['Mux/' num2str(nnn)])
      |     end
      |     
      | set_param(BusSel,'OutputSignals',outsig);
      | set_param(BusMux,'Inputs',num2str(length(Inputs)))
      | 
      | 
      | 
      |     
      |     for nnn = 1:length(Inputs)
      |         add_line([CurrentSys '/' blockName],['BusSelector/' num2str(nnn)],['Mux/' num2str(nnn)])
      |     end
  DLLSimulationStep : MATLABFcn  MATLABFcn=DLLSimStep(u,DLLSim.nDT)  OutputDimensions=DLLSim.nOuputs  SampleTime=dt
  Vector to Bus : Subsystem  Commented=on  mask{Nsigs=DLLSim.nOuputs}
      mask prompts: Nsigs "Signal Length"
  Vector to Bus v16_ : Subsystem  Variant=on
  SimOutputBus : Outport
  wires:
  Bus to Vector/1 -> DLLSimulationStep/1
  DLLSimulationStep/1 -> Vector to Bus v16_/1(In1)
  Vector to Bus v16_/1(Out1) -> SimOutputBus/1
  SimInputBus/1 -> Bus to Vector/1

== system Lib_Piccolo/A//C Dynamics/Gust Wind Input1 ==
  BA Sim Input IN : Inport
  Trigger : Inport  Port=2
  Gust Wind Model : Subsystem  VariantControl="GustType ~= \"NONE\""
  No Gust : Subsystem  VariantControl="GustType == \"NONE\""
  BA Sim Input OUT : Outport

== system Lib_Piccolo/A//C Dynamics/Jack Fail Flags ==
  In1 : Inport
  AoA Flag : Scope  Commented=on
  Bus Selector15 : BusSelector  OutputSignals=TASKts,AlphaDeg,NzG,AftFlapBDriveDeg,BetaDeg
  Constant : Constant  Value=m
  Constant1 : Constant  Value=-2
  Constant2 : Constant  Value=8
  Constant3 : Constant  Value=nMin_User
  Constant4 : Constant  Value=nMax_User
  Constant5 : Constant  Value=-ElevatorMax
  Constant6 : Constant  Value=ElevatorMax
  Divide : Product  Inputs=**
  Divide1 : Product  Inputs=*/
  Elevator Saturation Flag : Scope  Commented=on
  Gain3 : Gain  Gain=1.2
  Gain7 : Gain  Gain=0.99
  Gain8 : Gain  Gain=0.99
  GreaterThanOrEqual : RelationalOperator  Operator=<=  OutDataTypeStr=boolean  RndMeth=Simplest
  Knots to m/s1 : Gain  Gain=0.51444
  Less Than : RelationalOperator  Operator=<=  OutDataTypeStr=boolean  RndMeth=Simplest
  Less Than1 : RelationalOperator  OutDataTypeStr=boolean  RndMeth=Simplest
  Less Than2 : RelationalOperator  Operator=<=  OutDataTypeStr=boolean  RndMeth=Simplest
  Less Than3 : RelationalOperator  OutDataTypeStr=boolean  RndMeth=Simplest
  Less Than4 : RelationalOperator  Operator=<=  OutDataTypeStr=boolean  RndMeth=Simplest
  Less Than5 : RelationalOperator  OutDataTypeStr=boolean  RndMeth=Simplest
  "Load Factor Flag " : Scope  Commented=on
  OR : Logic  Operator=OR  IconShape=distinctive  AllPortsSameDT=off  OutDataTypeStr=boolean
  OR1 : Logic  Operator=OR  IconShape=distinctive  AllPortsSameDT=off  OutDataTypeStr=boolean
  OR2 : Logic  Operator=OR  IconShape=distinctive  AllPortsSameDT=off  OutDataTypeStr=boolean
  Sqrt : Sqrt  SaturateOnIntegerOverflow=on
  Square : Math  Operator=square  SaturateOnIntegerOverflow=on
  TAS Flag : Scope  Commented=on
  Terminator12 : Terminator
  Terminator13 : Terminator
  gain : Gain
  gain1 : Gain
  kg : Constant  Value=180
  m/s : Constant  Value=31
  wires:
  Divide1/1 -> Divide/2
  Constant6/1 -> Gain8/1
  Constant4/1 -> Less Than3/2
  Less Than5/1 -> OR2/2
  Bus Selector15/3 -> Less Than3/1, Less Than2/1  "<NzG>"
  Bus Selector15/2 -> gain/1, Less Than1/1, Less Than/1  "<AlphaDeg>"
  Gain8/1 -> Less Than5/2
  Less Than4/1 -> OR2/1
  OR2/1 -> Elevator Saturation Flag/1  "Flag_ElevatorSaturation"
  Less Than2/1 -> OR1/1
  Constant2/1 -> Less Than1/2
  Constant1/1 -> Less Than/2
  Gain7/1 -> Less Than4/2
  Less Than/1 -> OR/1
  Bus Selector15/1 -> Knots to m/s1/1  "<TASKts>"
  Constant/1 -> Divide/1
  Knots to m/s1/1 -> GreaterThanOrEqual/1  "Sim.TAS"
  Bus Selector15/4 -> Less Than5/1, Less Than4/1  "<AftFlapBDriveDeg>"
  m/s/1 -> Square/1
  Less Than3/1 -> OR1/2
  Less Than1/1 -> OR/2
  Gain3/1 -> GreaterThanOrEqual/2  "V_min"
  GreaterThanOrEqual/1 -> TAS Flag/1  "Flag_TAS"
  Bus Selector15/5 -> gain1/1  "<BetaDeg>"
  Square/1 -> Divide1/1
  OR1/1 -> "Load Factor Flag "/1  "Flag_LoadFactor"
  kg/1 -> Divide1/2
  Sqrt/1 -> Gain3/1  "V_stall"
  OR/1 -> AoA Flag/1  "Flag_AoA"
  Divide/1 -> Sqrt/1
  Constant5/1 -> Gain7/1
  gain/1 -> Terminator12/1  "Sim.AlphaDeg"
  gain1/1 -> Terminator13/1  "Sim.BetaDeg"
  Constant3/1 -> Less Than2/2
  In1/1 -> Bus Selector15/1
